simulink model "emso4"  (Simulink 7.1)
settings: Solver=ode4  StartTime=0.0  StopTime=5  RelTol=1e-3
settings Model: Creator=lades  LastModifiedBy=Administrator
settings DataIOCC: ExternalInput=Az

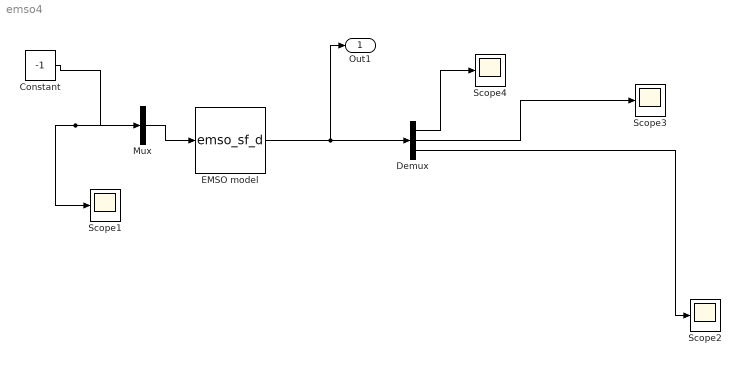
== system emso4 ==
  Constant : Constant  Value=-1  OutDataType=sfix(16)  OutScaling=2^0
  Demux : Demux  Outputs=3
  EMSO model : S-Function  FunctionName=emso_sf_d  Parameters='Problem_2F.ems',1,3,0.05  EnableBusSupport=off
  Mux : Mux  Inputs=1
  Scope{1..4} (4 alike) : Scope
      Scope1 settings: TimeRange=2  YMin=4.008258966500001  YMax=4.008258969500001
      Scope2 settings: TimeRange=5  YMin=0  YMax=45
      Scope3 settings: TimeRange=5  YMin=0  YMax=45  SaveName=ScopeData2
      Scope4 settings: TimeRange=5  YMin=0  YMax=45  SaveName=ScopeData3
  Out1 : Outport  OutDataType=sfix(16)  OutScaling=2^0
  wires:
  EMSO model/1 -> Demux/1, Out1/1
  Mux/1 -> EMSO model/1
  Constant/1 -> Mux/1, Scope1/1
  Demux/3 -> Scope2/1
  Demux/2 -> Scope3/1
  Demux/1 -> Scope4/1
